simulink model "SixDOFSim"  (R2026b)
settings: Solver=VariableStepAuto  StopTime=400
values from neighbouring files (symbols this model uses):
  A = [A_1 zeros(n/2,n/2);zeros(n/2,n/2) A_2]    [defineABC.m]    (also in implicit_linmod.m = -inv(E)*A_prime; nonlinear_6DOF.m = q_d*S*CA; normieren.m = Tx\A*Tx)
  B = [B_1, zeros(n/2,m/2);zeros(n/2,m/2), B_2]    [defineABC.m]    (also in implicit_linmod.m = -inv(E)*B_prime; normieren.m = Tx\B*Tu)
  C = zeros(m,n)    [defineABC.m]    (also in normieren.m = (Ty\C*Tx))
  eta_max = 10*pi/180    (= 0.174532925199)    [SixDOFModel.m]
  eta_min = - 25*pi/180    (= -0.436332312999)    [SixDOFModel.m]
  F = -inv(C*(Ak\B))    [SixDOFModel.m]    (also in coupling_controller.m = Kopt{end}; implicit_linmod.m = feval(fun, dX_ap, X_ap, U_minus))
  I_inv = inv(I)    [initializeParameters.m]
  K = lqr(sys_ol,Q,R)    [SixDOFModel.m]
  latlon_init = [0;0]    [SixDOFModel.m]
  m = size(B_1,2) + size(B_2,2)    [defineABC.m]    (also in implicit_linmod.m = length(U_ap); initializeParameters.m = 120000)
  n = size(A_1,1) +size(A_2,2)    [defineABC.m]    (also in implicit_linmod.m = length(X_ap); normieren.m = size(A,2))
  Omega_init_1 = [0;0;0]    [SixDOFModel.m]
  Omega_init_2 = [0;0;0]    [SixDOFModel.m]
  P_e_init_1 = [0;0;-h_init_1]    [SixDOFModel.m]
  P_e_init_2 = [0;0;-h_init_2]    [SixDOFModel.m]
  Phi_init_1 = [0;0;0]    [SixDOFModel.m]
  Phi_init_2 = [0;0;0]    [SixDOFModel.m]
  sigmaf_max = 10*pi/180    (= 0.174532925199)    [SixDOFModel.m]
  sigmaf_min = 0.5*pi/180    (= 0.00872664625997)    [SixDOFModel.m]
  U_ap = [U_ap_1;U_ap_2]    [SixDOFModel.m]    (also in trimValues.m = Z_ap(11:14))
  U_test = [-0.12;1;0;0;-0.1;1;0;0]    [SixDOFModel.m]
  V_init_1 = [200;0;0]    [SixDOFModel.m]
  V_init_2 = [220;0;0]    [SixDOFModel.m]
  W_ap = [X_ap_1(1); X_ap_2(1); 0; 0; X_ap_1(10); X_ap_2(10); 0; 0]    [SixDOFModel.m]
  X_ap = [X_ap_1;X_ap_2]    [SixDOFModel.m]    (also in trimValues.m = Z_ap(1:10))
  X_init = [X_init_1;X_init_2]    [SixDOFModel.m]
  xi_max = 25*pi/180    (= 0.436332312999)    [SixDOFModel.m]
  xi_min = - xi_max    (= -0.436332312999)    [SixDOFModel.m]
  zita_max = 30*pi/180    (= 0.523598775598)    [SixDOFModel.m]
  zita_min = - zita_max    (= -0.523598775598)    [SixDOFModel.m]
undefined symbols (not defined in the file or in its folder): Earth, globalParameters, nonlinear_6DOF, WGS84
libraries: aerolibfltsims x38, aerolibtransform2 x6, aerolibwind2 x2, simulink x2, aerolibatmos2 x2
(part 1 of 3)
settings Model: Creator=teteu  LastModifiedBy=zhang
settings SolverCC: ZeroCrossAlgorithm=Adaptive
settings DebuggingCC: IgnoredZcDiagnostic=none  UnderSpecifiedDimensionMsg=warning
settings RTWCC: DLArmComputeVersion=19.05
settings SimscapeCC: SimscapeUseEnergyAccounting=off

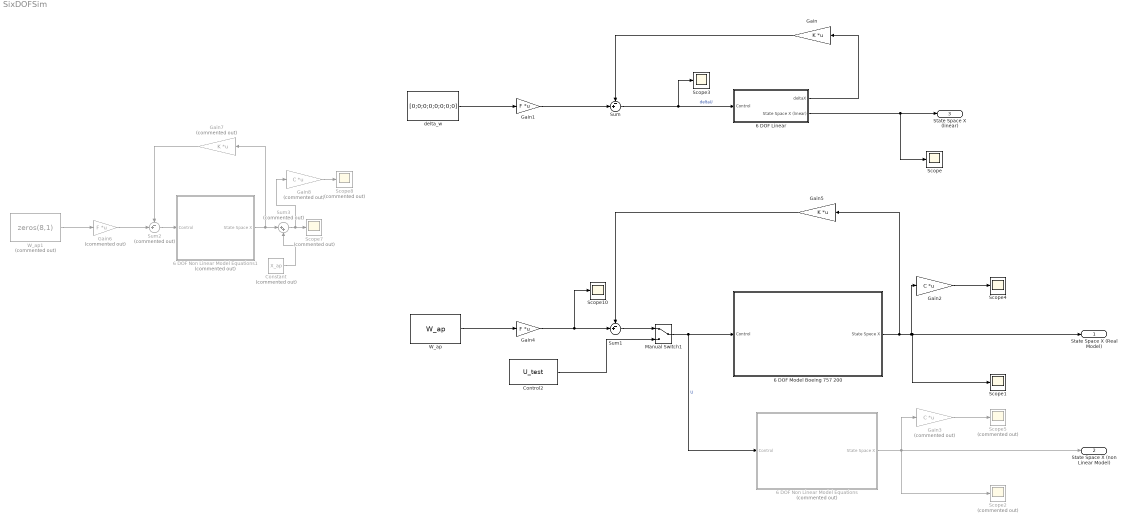
== system SixDOFSim ==
  6 DOF Linear : Subsystem
  6 DOF Model Boeing 757 200 : Subsystem
      mask Display: image('Eastern_Airlines_Boeing_757-225_N523EA_March_1990_DCW_4974892113-624x422.jpg'); % Use "Edit Image" on toolstrip to change.
  6 DOF Non Linear Model Equations : Subsystem  Commented=on
      mask Display: image('491461_1_En_8_Fig2_HTML.png');
  6 DOF Non Linear Model Equations1 : Subsystem  Commented=on
      mask Display: image('491461_1_En_8_Fig2_HTML.png');
  Constant : Constant  Commented=on  Value=X_ap
  Control2 : Constant  Value=U_test
  Gain : Gain  Gain=K  Multiplication=Matrix(K*u)
  Gain1 : Gain  Gain=F  Multiplication=Matrix(K*u)
  Gain2 : Gain  Gain=C  Multiplication=Matrix(K*u)
  Gain3 : Gain  Commented=on  Gain=C  Multiplication=Matrix(K*u)
  Gain4 : Gain  Gain=F  Multiplication=Matrix(K*u)
  Gain5 : Gain  Gain=K  Multiplication=Matrix(K*u)
  Gain6 : Gain  Commented=on  Gain=F  Multiplication=Matrix(K*u)
  Gain7 : Gain  Commented=on  Gain=K  Multiplication=Matrix(K*u)
  Gain8 : Gain  Commented=on  Gain=C  Multiplication=Matrix(K*u)
  Manual Switch1 : ManualSwitch
  Scope{,1,3..4,10} (5 alike) : Scope
      Scope settings: ActiveDisplayYMinimum=7776.65926  ActiveDisplayYMaximum=8271.84202
      Scope1 settings: ActiveDisplayYMinimum=-9243.3104191158855  ActiveDisplayYMaximum=16255.898989328776  DataLoggingVariableName=ScopeData2
      Scope10 settings: ActiveDisplayYMinimum=-20.03565  ActiveDisplayYMaximum=4.07413  DataLoggingVariableName=ScopeData6
      Scope3 settings: ActiveDisplayYMinimum=-0.10509  ActiveDisplayYMaximum=0.02343  DataLoggingVariableName=ScopeData4
      Scope4 settings: ActiveDisplayYMinimum=-2103.5512790095572  ActiveDisplayYMaximum=10071.687214697096
  Scope{2,5,7..8} (4 alike) : Scope  Commented=on
      Scope2 settings: ActiveDisplayYMinimum=-1023.1359  ActiveDisplayYMaximum=9013.89641  DataLoggingVariableName=ScopeData3
      Scope5 settings: ActiveDisplayYMinimum=-1001.29057  ActiveDisplayYMaximum=9011.46915  DataLoggingVariableName=ScopeData2
      Scope7 settings: ActiveDisplayYMinimum=-11.89027  ActiveDisplayYMaximum=4.789  DataLoggingVariableName=ScopeData4
      Scope8 settings: ActiveDisplayYMinimum=-111.74089  ActiveDisplayYMaximum=88.33649  DataLoggingVariableName=ScopeData5
  Sum : Sum  Inputs=-+|
  Sum1 : Sum  Inputs=-+|
  Sum2 : Sum  Commented=on  Inputs=-+|
  Sum3 : Sum  Commented=on  Inputs=|++
  W_ap : Constant  Value=W_ap
  W_ap1 : Constant  Commented=on  Value=zeros(8,1)
  delta_w : Constant  Value=[0;0;0;0;0;0;0;0]
  State Space X (Real Model) : Outport
  State Space X (non Linear Model) : Outport  Port=2
  State Space X (linear) : Outport  Port=3
  wires:
  Gain/1 -> Sum/1
  Sum/1 -> Scope3/1, 6 DOF Linear/1(Control)  "deltaU"
  6 DOF Linear/2(State Space X (linear)) -> Scope/1, State Space X (linear)/1
  6 DOF Model Boeing 757 200/1(State Spece X) -> Gain5/1, Gain2/1, Scope1/1, State Space X (Real Model)/1
  6 DOF Non Linear Model Equations/1(State Space X) -> Gain3/1, State Space X (non Linear Model)/1, Scope2/1
  delta_w/1 -> Gain1/1
  Gain1/1 -> Sum/2
  6 DOF Linear/1(deltaX) -> Gain/1
  Gain2/1 -> Scope4/1
  Gain3/1 -> Scope5/1
  W_ap/1 -> Gain4/1
  Gain4/1 -> Scope10/1, Sum1/2
  Gain5/1 -> Sum1/1
  Sum1/1 -> Manual Switch1/1
  Manual Switch1/1 -> 6 DOF Non Linear Model Equations/1(Control), 6 DOF Model Boeing 757 200/1(Control)  "U"
  6 DOF Non Linear Model Equations1/1(State Space X) -> Sum3/1, Gain7/1
  Sum2/1 -> 6 DOF Non Linear Model Equations1/1(Control)
  Gain7/1 -> Sum2/1
  Gain8/1 -> Scope8/1
  W_ap1/1 -> Gain6/1
  Gain6/1 -> Sum2/2
  Sum3/1 -> Gain8/1, Scope7/1
  Constant/1 -> Sum3/2
  Control2/1 -> Manual Switch1/2

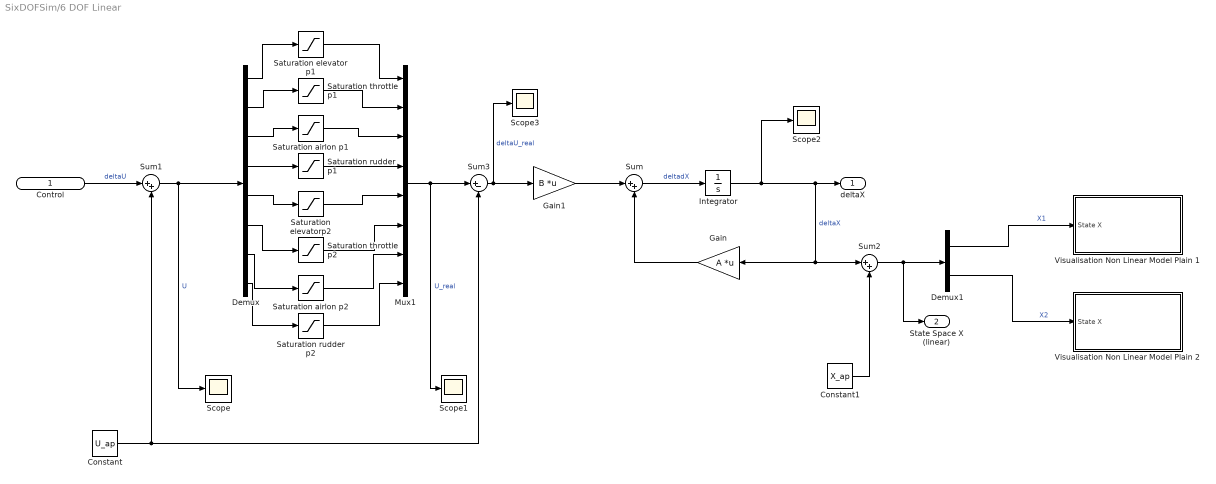
== system SixDOFSim/6 DOF Linear ==
  Control : Inport
  Constant : Constant  Value=U_ap
  Constant1 : Constant  Value=X_ap
  Demux : Demux  Outputs=8
  Demux1 : Demux  Outputs=2
  Gain : Gain  Gain=A  Multiplication=Matrix(K*u)
  Gain1 : Gain  Gain=B  Multiplication=Matrix(K*u)
  Integrator : Integrator  InitialCondition=X_init-X_ap
  Mux1 : Mux  Inputs=8
  Saturation airlon p1 : Saturate  UpperLimit=xi_max  LowerLimit=xi_min
  Saturation airlon p2 : Saturate  UpperLimit=xi_max  LowerLimit=xi_min
  Saturation elevator p1 : Saturate  UpperLimit=eta_max  LowerLimit=eta_min
  Saturation elevatorp2 : Saturate  UpperLimit=eta_max  LowerLimit=eta_min
  Saturation rudder p1 : Saturate  UpperLimit=zita_max  LowerLimit=zita_min
  Saturation rudder p2 : Saturate  UpperLimit=zita_max  LowerLimit=zita_min
  Saturation throttle p1 : Saturate  UpperLimit=sigmaf_max  LowerLimit=sigmaf_min
  Saturation throttle p2 : Saturate  UpperLimit=sigmaf_max  LowerLimit=sigmaf_min
  Scope{,1..3} (4 alike) : Scope
      Scope settings: ActiveDisplayYMinimum=-0.19857  ActiveDisplayYMaximum=0.43595  DataLoggingVariableName=ScopeData2
      Scope1 settings: ActiveDisplayYMinimum=-0.34609  ActiveDisplayYMaximum=0.23238
      Scope2 settings: ActiveDisplayYMinimum=-0.60126  ActiveDisplayYMaximum=0.68136
      Scope3 settings: ActiveDisplayYMinimum=-0.00918  ActiveDisplayYMaximum=0.00122  DataLoggingVariableName=ScopeData2
  Sum : Sum  Inputs=|++
  Sum1 : Sum  Inputs=|++
  Sum2 : Sum  Inputs=|++
  Sum3 : Sum  Inputs=|+-
  Visualisation Non Linear Model Plain 1 : Subsystem
  Visualisation Non Linear Model Plain 2 : Subsystem
  deltaX : Outport
  State Space X (linear) : Outport  Port=2
  wires:
  Gain1/1 -> Sum/1
  Sum/1 -> Integrator/1  "deltadX"
  Gain/1 -> Sum/2
  Demux/2 -> Saturation throttle p1/1
  Demux/3 -> Saturation airlon p1/1
  Demux/1 -> Saturation elevator p1/1
  Saturation elevator p1/1 -> Mux1/1
  Saturation throttle p1/1 -> Mux1/2
  Saturation airlon p1/1 -> Mux1/3
  Saturation rudder p1/1 -> Mux1/4
  Demux/4 -> Saturation rudder p1/1
  Control/1 -> Sum1/1  "deltaU"
  Constant/1 -> Sum1/2, Sum3/2
  Integrator/1 -> Scope2/1, deltaX/1, Sum2/1, Gain/1  "deltaX"
  Demux1/1 -> Visualisation Non Linear Model Plain 1/1(State X)  "X1"
  Demux1/2 -> Visualisation Non Linear Model Plain 2/1(State X)  "X2"
  Demux/5 -> Saturation elevatorp2/1
  Saturation elevatorp2/1 -> Mux1/5
  Demux/6 -> Saturation throttle p2/1
  Demux/7 -> Saturation airlon p2/1
  Saturation throttle p2/1 -> Mux1/6
  Saturation airlon p2/1 -> Mux1/7
  Demux/8 -> Saturation rudder p2/1
  Saturation rudder p2/1 -> Mux1/8
  Sum1/1 -> Demux/1, Scope/1  "U"
  Mux1/1 -> Sum3/1, Scope1/1  "U_real"
  Sum2/1 -> State Space X (linear)/1, Demux1/1
  Constant1/1 -> Sum2/2
  Sum3/1 -> Scope3/1, Gain1/1  "deltaU_real"

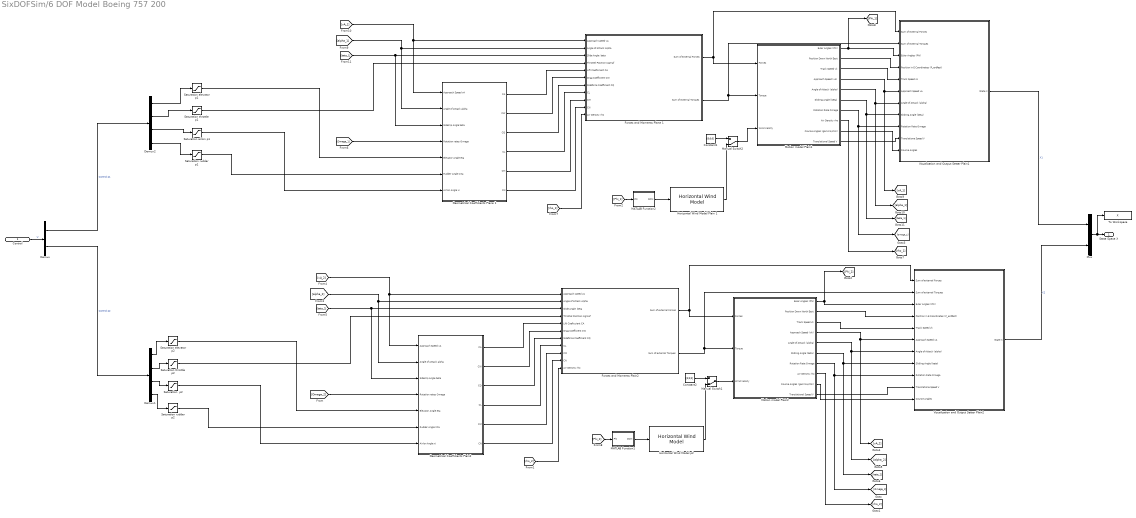
== system SixDOFSim/6 DOF Model Boeing 757 200 ==
  Control : Inport
  Constant1 : Constant  Value=[0;0;0]
  Constant2 : Constant  Value=[0;0;0]
  Demux : Demux  Outputs=2
  Demux1 : Demux
  Demux2 : Demux
  Forces and Moments Plain2 : Subsystem
  Forces and Moments Plane 1 : Subsystem
  Geometrical Coefficients Plain2 : Subsystem
  Geometrical Coefficients Plane 1 : Subsystem
  Horizontal Wind Model Plain 1 : aerolibwind2/Horizontal Wind Model  units=Metric (MKS)  Vw_source=Internal  Vwind=15  W_source=Internal  Wdeg=0
  Horizontal Wind Model p2 : aerolibwind2/Horizontal Wind Model  units=Metric (MKS)  Vw_source=Internal  Vwind=15  W_source=Internal  Wdeg=0
  MATLAB Function1 : MATLAB Function  TreatAsAtomicUnit=on
  MATLAB Function2 : MATLAB Function  TreatAsAtomicUnit=on
  Manual Switch1 : ManualSwitch  CurrentSetting=0
  Manual Switch2 : ManualSwitch  CurrentSetting=0
  Motion model Plain1 : Subsystem
  "Motion model Plain2 " : Subsystem
  Mux : Mux  Inputs=2
  Saturation  p2 : Saturate  UpperLimit=xi_max  LowerLimit=xi_min
  Saturation airlon p1 : Saturate  UpperLimit=xi_max  LowerLimit=xi_min
  Saturation elevator p1 : Saturate  UpperLimit=eta_max  LowerLimit=eta_min
  Saturation elevator p2 : Saturate  UpperLimit=eta_max  LowerLimit=eta_min
  Saturation rudder p1 : Saturate  UpperLimit=zita_max  LowerLimit=zita_min
  Saturation rudder p2 : Saturate  UpperLimit=zita_max  LowerLimit=zita_min
  Saturation throttle p1 : Saturate  UpperLimit=sigmaf_max  LowerLimit=sigmaf_min
  Saturation throttle p2 : Saturate  UpperLimit=sigmaf_max  LowerLimit=sigmaf_min
  To Workspace : ToWorkspace  VariableName=X  SaveFormat=Timeseries  SampleTime=-1
  Visualization and Output Setter Plain1 : Subsystem
  Visualization and Output Setter Plain2 : Subsystem
  State Spece X : Outport
  wires:
  "Motion model Plain2 "/7(Rotation Rate Omega) -> [Omega_2], Visualization and Output Setter Plain2/9(Rotation Rate Omega)
  "Motion model Plain2 "/3(Track Speed vk) -> Visualization and Output Setter Plain2/5(Track Speed vk)
  Visualization and Output Setter Plain2/1(State X) -> Mux/2  "X2"
  "Motion model Plain2 "/6(Slidiing Angle (beta)) -> [beta_2], Visualization and Output Setter Plain2/8(Slidiing Angle (beta))
  Forces and Moments Plain2/2(Sum of external Torques) -> Visualization and Output Setter Plain2/2(Sum of external Torques), "Motion model Plain2 "/2(Torque)
  [alpha_2] -> Geometrical Coefficients Plain2/2(Angle of Attack alpha), Forces and Moments Plain2/2(Angle of Attack Alpha)
  "Motion model Plain2 "/4(Approach Speed (vA)) -> [vA_2], Visualization and Output Setter Plain2/6(Approach Speed vA)
  Geometrical Coefficients Plain2/4(CL) -> Forces and Moments Plain2/8(CL)
  Geometrical Coefficients Plain2/1(CA) -> Forces and Moments Plain2/5(Lift Coeficcient CA)
  Forces and Moments Plain2/1(Sum of external Forces) -> Visualization and Output Setter Plain2/1(Sum of external Forces), "Motion model Plain2 "/1(Forces)
  "Motion model Plain2 "/5(Angle of Attack (alpha)) -> [alpha_2], Visualization and Output Setter Plain2/7(Angle of Attack (alpha))
  "Motion model Plain2 "/2(Position Down North East) -> Visualization and Output Setter Plain2/4(Position in E Coordinates (P_erdfest))
  "Motion model Plain2 "/1(Euler Angles (Phi)) -> [Phi_2], Visualization and Output Setter Plain2/3(Euler Angles (Phi))
  [vA_2] -> Geometrical Coefficients Plain2/1(Approach Speed vA), Forces and Moments Plain2/1(Approach speed vA)
  Geometrical Coefficients Plain2/5(CM) -> Forces and Moments Plain2/9(CM)
  Saturation  p2/1 -> Geometrical Coefficients Plain2/7(Airlon Angle xi)
  [Omega_2] -> Geometrical Coefficients Plain2/4(Rotation rates Omega)
  Saturation throttle p2/1 -> Forces and Moments Plain2/4(Throttel Position sigmaf)
  [beta_2] -> Geometrical Coefficients Plain2/3(Sideslip Angle beta), Forces and Moments Plain2/3(Slide Angle  beta)
  Geometrical Coefficients Plain2/6(CN) -> Forces and Moments Plain2/10(CN)
  "Motion model Plain2 "/8(Air Density rho) -> [rho_2]
  [rho_2] -> Forces and Moments Plain2/11(Air Density rho)
  Saturation elevator p2/1 -> Geometrical Coefficients Plain2/5(Elevator Angle eta)
  Saturation rudder p2/1 -> Geometrical Coefficients Plain2/6(Rudder Angle zita)
  Geometrical Coefficients Plain2/3(CQ) -> Forces and Moments Plain2/7(Sideforce Coefficient CQ)
  Geometrical Coefficients Plain2/2(CW) -> Forces and Moments Plain2/6(Drag Coefficient CW)
  Demux1/2 -> Saturation throttle p2/1
  Demux1/3 -> Saturation  p2/1
  Demux1/1 -> Saturation elevator p2/1
  Demux1/4 -> Saturation rudder p2/1
  "Motion model Plain2 "/9("Course Angles (gamma;chsi) ") -> Visualization and Output Setter Plain2/11("Course Angles ")
  "Motion model Plain2 "/10(Translational Speed V) -> Visualization and Output Setter Plain2/10(Translationa Speed V)
  Manual Switch1/1 -> "Motion model Plain2 "/3(Wind Veloity)
  Saturation rudder p1/1 -> Geometrical Coefficients Plane 1/6(Rudder Angle zita)
  Motion model Plain1/5(Angle of Attack (alpha)) -> [alpha_1], Visualization and Output Setter Plain1/7(Angle of Attack (alpha))
  Motion model Plain1/1(Euler Angles (Phi)) -> [Phi_1], Visualization and Output Setter Plain1/3(Euler Angles (Phi))
  Forces and Moments Plane 1/1(Sum of external Forces) -> Visualization and Output Setter Plain1/1(Sum of external Forces), Motion model Plain1/1(Forces)
  Motion model Plain1/10(Translational Speed V) -> Visualization and Output Setter Plain1/10(Translationa Speed V)
  [Omega_1] -> Geometrical Coefficients Plane 1/4(Rotation rates Omega)
  Geometrical Coefficients Plane 1/2(CW) -> Forces and Moments Plane 1/6(Drag Coefficient CW)
  [beta_1] -> Geometrical Coefficients Plane 1/3(Sideslip Angle beta), Forces and Moments Plane 1/3(Slide Angle  beta)
  Geometrical Coefficients Plane 1/3(CQ) -> Forces and Moments Plane 1/7(Sideforce Coefficient CQ)
  Geometrical Coefficients Plane 1/4(CL) -> Forces and Moments Plane 1/8(CL)
  Saturation airlon p1/1 -> Geometrical Coefficients Plane 1/7(Airlon Angle xi)
  Geometrical Coefficients Plane 1/5(CM) -> Forces and Moments Plane 1/9(CM)
  Motion model Plain1/4(Approach Speed (vA)) -> [vA_1], Visualization and Output Setter Plain1/6(Approach Speed vA)
  Demux2/3 -> Saturation airlon p1/1
  [vA_1] -> Geometrical Coefficients Plane 1/1(Approach Speed vA), Forces and Moments Plane 1/1(Approach speed vA)
  Saturation throttle p1/1 -> Forces and Moments Plane 1/4(Throttel Position sigmaf)
  Demux2/1 -> Saturation elevator p1/1
  Motion model Plain1/2(Position Down North East) -> Visualization and Output Setter Plain1/4(Position in E Coordinates (P_erdfest))
  Geometrical Coefficients Plane 1/1(CA) -> Forces and Moments Plane 1/5(Lift Coeficcient CA)
  Demux2/2 -> Saturation throttle p1/1
  Motion model Plain1/8(Air Density rho) -> [rho_1]
  [rho_1] -> Forces and Moments Plane 1/11(Air Density rho)
  Motion model Plain1/6(Slidiing Angle (beta)) -> [beta_1], Visualization and Output Setter Plain1/8(Slidiing Angle (beta))
  Demux2/4 -> Saturation rudder p1/1
  Motion model Plain1/9("Course Angles (gamma;chsi) ") -> Visualization and Output Setter Plain1/11("Course Angles ")
  Motion model Plain1/7(Rotation Rate Omega) -> [Omega_1], Visualization and Output Setter Plain1/9(Rotation Rate Omega)
  Saturation elevator p1/1 -> Geometrical Coefficients Plane 1/5(Elevator Angle eta)
  Forces and Moments Plane 1/2(Sum of external Torques) -> Visualization and Output Setter Plain1/2(Sum of external Torques), Motion model Plain1/2(Torque)
  [alpha_1] -> Geometrical Coefficients Plane 1/2(Angle of Attack alpha), Forces and Moments Plane 1/2(Angle of Attack Alpha)
  Geometrical Coefficients Plane 1/6(CN) -> Forces and Moments Plane 1/10(CN)
  Motion model Plain1/3(Track Speed vk) -> Visualization and Output Setter Plain1/5(Track Speed vk)
  Visualization and Output Setter Plain1/1(State X) -> Mux/1  "X1"
  [Phi_2] -> MATLAB Function1/1(Phi)
  Horizontal Wind Model p2/1 -> Manual Switch1/2
  MATLAB Function1/1(DCM) -> Horizontal Wind Model p2/1
  Control/1 -> Demux/1  "U"
  Demux/1 -> Demux2/1  "Control p1"
  Demux/2 -> Demux1/1  "Control p2"
  Constant2/1 -> Manual Switch1/1
  MATLAB Function2/1(DCM) -> Horizontal Wind Model Plain 1/1
  [Phi_1] -> MATLAB Function2/1(Phi)
  Constant1/1 -> Manual Switch2/1
  Horizontal Wind Model Plain 1/1 -> Manual Switch2/2
  Manual Switch2/1 -> Motion model Plain1/3(Wind Veloity)
  Mux/1 -> To Workspace/1, State Spece X/1

== system SixDOFSim/6 DOF Non Linear Model Equations ==
  Control : Inport
  Demux : Demux
  Demux1 : Demux
  Demux2 : Demux  Outputs=2
  Integrator : Integrator  InitialCondition=X_init(1:n/2)
  Integrator1 : Integrator  InitialCondition=X_init(1+n/2:end)
  Model of the Plain Equations 1 : MATLABFcn  MATLABFcn=nonlinear_6DOF(u(1:10),u(11:14),u(15))
  Model of the Plain Equations 2 : MATLABFcn  MATLABFcn=nonlinear_6DOF(u(1:10),u(11:14),u(15))
  Mux : Mux  Inputs=3
  Mux1 : Mux
  Mux2 : Mux  Inputs=3
  Mux3 : Mux
  Mux4 : Mux  Inputs=2
  Mux5 : Mux  Inputs=2
  Saturation airlon p1 : Saturate  UpperLimit=xi_max  LowerLimit=xi_min
  Saturation airlonp2 : Saturate  UpperLimit=xi_max  LowerLimit=xi_min
  Saturation elevator p1 : Saturate  UpperLimit=eta_max  LowerLimit=eta_min
  Saturation elevator p2 : Saturate  UpperLimit=eta_max  LowerLimit=eta_min
  Saturation rudder p1 : Saturate  UpperLimit=zita_max  LowerLimit=zita_min
  Saturation rudder p2 : Saturate  UpperLimit=zita_max  LowerLimit=zita_min
  Saturation throttle p1 : Saturate  UpperLimit=sigmaf_max  LowerLimit=sigmaf_min
  Saturation throttle p2 : Saturate  UpperLimit=sigmaf_max  LowerLimit=sigmaf_min
  Scope : Scope
      settings: ActiveDisplayYMinimum=-0.40615  ActiveDisplayYMaximum=0.92239  DataLoggingVariableName=ScopeData3
  Scope1 : Scope
      settings: ActiveDisplayYMinimum=-0.28294  ActiveDisplayYMaximum=0.22359  DataLoggingVariableName=ScopeData4
  Select Plain 1 : Constant
  Select Plain 2 : Constant  Value=2
  Visualisation Non Linear Model 1 : Subsystem
  Visualisation Non Linear Model 2 : Subsystem  Commented=on
  State Space X : Outport
  wires:
  Model of the Plain Equations 1/1 -> Integrator/1  "dX"
  Integrator/1 -> Visualisation Non Linear Model 1/1(State X), Mux/1, Mux4/1  "X1"
  Mux/1 -> Model of the Plain Equations 1/1
  Demux/1 -> Saturation elevator p1/1
  Demux/2 -> Saturation throttle p1/1
  Demux/3 -> Saturation airlon p1/1
  Demux/4 -> Saturation rudder p1/1
  Saturation elevator p1/1 -> Mux1/1
  Saturation throttle p1/1 -> Mux1/2
  Saturation airlon p1/1 -> Mux1/3
  Saturation rudder p1/1 -> Mux1/4
  Mux1/1 -> Mux5/1, Mux/2  "Control Plain 1"
  Mux2/1 -> Model of the Plain Equations 2/1
  Integrator1/1 -> Visualisation Non Linear Model 2/1(State X), Mux4/2, Mux2/1  "X2"
  Mux3/1 -> Mux2/2, Mux5/2  "Control P2"
  Saturation rudder p2/1 -> Mux3/4
  Saturation throttle p2/1 -> Mux3/2
  Saturation elevator p2/1 -> Mux3/1
  Demux2/2 -> Demux1/1
  Saturation airlonp2/1 -> Mux3/3
  Demux1/1 -> Saturation elevator p2/1
  Demux1/3 -> Saturation airlonp2/1
  Demux1/4 -> Saturation rudder p2/1
  Demux1/2 -> Saturation throttle p2/1
  Model of the Plain Equations 2/1 -> Integrator1/1  "dX"
  Control/1 -> Scope/1, Demux2/1
  Demux2/1 -> Demux/1
  Mux4/1 -> State Space X/1
  Select Plain 1/1 -> Mux/3
  Select Plain 2/1 -> Mux2/3
  Mux5/1 -> Scope1/1

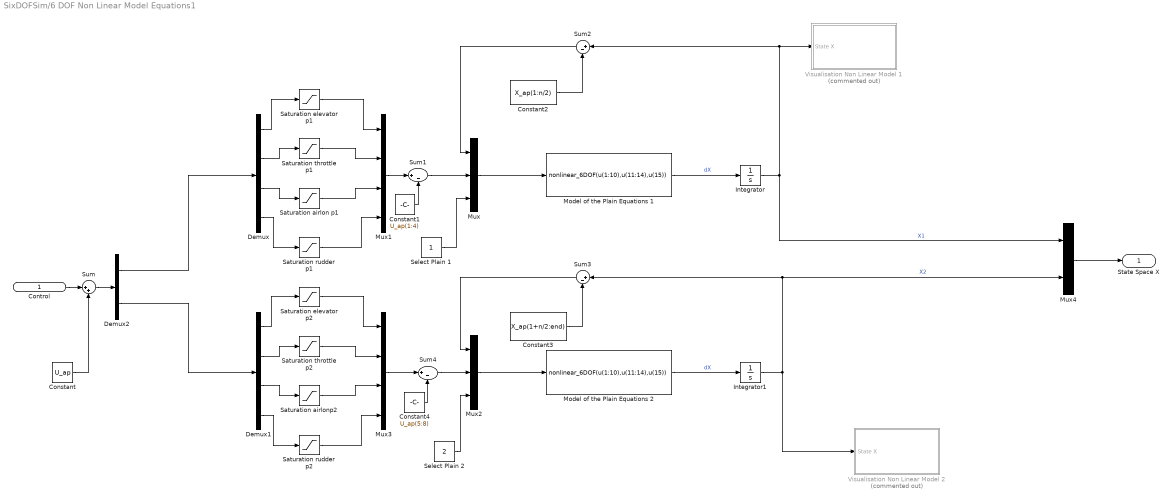
== system SixDOFSim/6 DOF Non Linear Model Equations1 ==
  Control : Inport
  Constant : Constant  Value=U_ap
  Constant1 : Constant  Value=U_ap(1:4)
  Constant2 : Constant  Value=X_ap(1:n/2)
  Constant3 : Constant  Value=X_ap(1+n/2:end)
  Constant4 : Constant  Value=U_ap(5:8)
  Demux : Demux
  Demux1 : Demux
  Demux2 : Demux  Outputs=2
  Integrator : Integrator  InitialCondition=X_init(1:n/2)-X_ap(1:n/2)
  Integrator1 : Integrator  InitialCondition=X_init(1+n/2:end)-X_ap(1+n/2:end)
  Model of the Plain Equations 1 : MATLABFcn  MATLABFcn=nonlinear_6DOF(u(1:10),u(11:14),u(15))
  Model of the Plain Equations 2 : MATLABFcn  MATLABFcn=nonlinear_6DOF(u(1:10),u(11:14),u(15))
  Mux : Mux  Inputs=3
  Mux1 : Mux
  Mux2 : Mux  Inputs=3
  Mux3 : Mux
  Mux4 : Mux  Inputs=2
  Saturation airlon p1 : Saturate  UpperLimit=xi_max  LowerLimit=xi_min
  Saturation airlonp2 : Saturate  UpperLimit=xi_max  LowerLimit=xi_min
  Saturation elevator p1 : Saturate  UpperLimit=eta_max  LowerLimit=eta_min
  Saturation elevator p2 : Saturate  UpperLimit=eta_max  LowerLimit=eta_min
  Saturation rudder p1 : Saturate  UpperLimit=zita_max  LowerLimit=zita_min
  Saturation rudder p2 : Saturate  UpperLimit=zita_max  LowerLimit=zita_min
  Saturation throttle p1 : Saturate  UpperLimit=sigmaf_max  LowerLimit=sigmaf_min
  Saturation throttle p2 : Saturate  UpperLimit=sigmaf_max  LowerLimit=sigmaf_min
  Select Plain 1 : Constant
  Select Plain 2 : Constant  Value=2
  Sum : Sum  Inputs=|++
  Sum{1..4} (4 alike) : Sum  Inputs=|+-
  Visualisation Non Linear Model 1 : Subsystem  Commented=on
  Visualisation Non Linear Model 2 : Subsystem  Commented=on
  State Space X : Outport
  wires:
  Model of the Plain Equations 1/1 -> Integrator/1  "dX"
  Integrator/1 -> Visualisation Non Linear Model 1/1(State X), Sum2/1, Mux4/1  "X1"
  Mux/1 -> Model of the Plain Equations 1/1
  Demux/1 -> Saturation elevator p1/1
  Demux/2 -> Saturation throttle p1/1
  Demux/3 -> Saturation airlon p1/1
  Demux/4 -> Saturation rudder p1/1
  Saturation elevator p1/1 -> Mux1/1
  Saturation throttle p1/1 -> Mux1/2
  Saturation airlon p1/1 -> Mux1/3
  Saturation rudder p1/1 -> Mux1/4
  Mux2/1 -> Model of the Plain Equations 2/1
  Integrator1/1 -> Visualisation Non Linear Model 2/1(State X), Mux4/2, Sum3/1  "X2"
  Saturation rudder p2/1 -> Mux3/4
  Saturation throttle p2/1 -> Mux3/2
  Saturation elevator p2/1 -> Mux3/1
  Demux2/2 -> Demux1/1
  Saturation airlonp2/1 -> Mux3/3
  Demux1/1 -> Saturation elevator p2/1
  Demux1/3 -> Saturation airlonp2/1
  Demux1/4 -> Saturation rudder p2/1
  Demux1/2 -> Saturation throttle p2/1
  Model of the Plain Equations 2/1 -> Integrator1/1  "dX"
  Demux2/1 -> Demux/1
  Mux4/1 -> State Space X/1
  Select Plain 1/1 -> Mux/3
  Select Plain 2/1 -> Mux2/3
  Sum/1 -> Demux2/1
  Control/1 -> Sum/1
  Constant/1 -> Sum/2
  Sum1/1 -> Mux/2
  Mux1/1 -> Sum1/1
  Constant1/1 -> Sum1/2
  Sum2/1 -> Mux/1
  Constant2/1 -> Sum2/2
  Constant3/1 -> Sum3/2
  Sum3/1 -> Mux2/1
  Sum4/1 -> Mux2/2
  Constant4/1 -> Sum4/2
  Mux3/1 -> Sum4/1

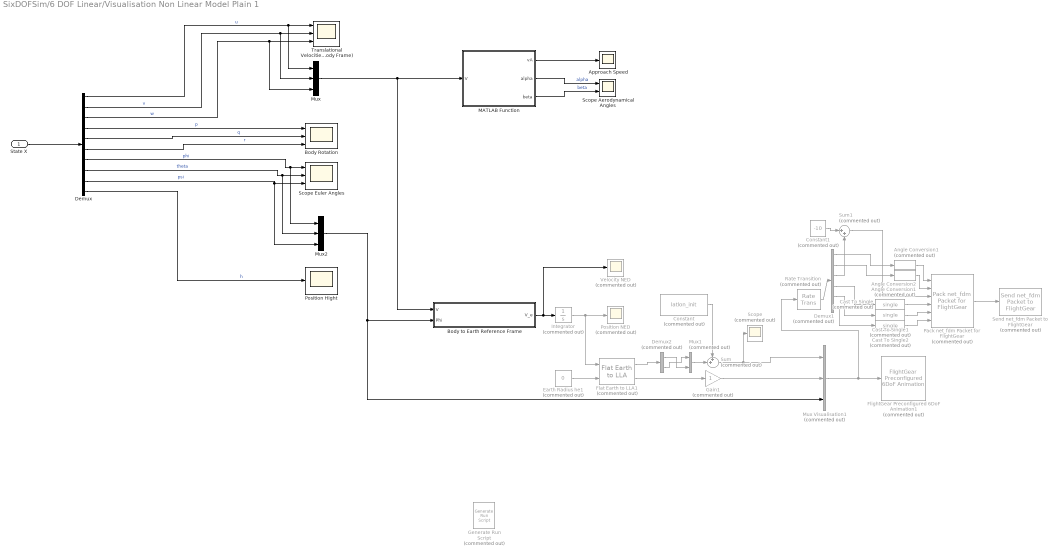
== system SixDOFSim/6 DOF Linear/Visualisation Non Linear Model Plain 1 ==
  State X : Inport
  Angle Conversion1 : aerolibfltsims/FlightGear Preconfigured 6DoF Animation/Angle Conversion1  Commented=on  SystemSampleTime=-1  VariantActivationTime=update diagram  Latency=0  AutoFrameSizeCalculation=off
  Angle Conversion2 : aerolibfltsims/FlightGear Preconfigured 6DoF Animation/Angle Conversion1  Commented=on  SystemSampleTime=-1  VariantActivationTime=update diagram  Latency=0  AutoFrameSizeCalculation=off
  Approach Speed : Scope
      settings: ActiveDisplayYMinimum=91.83935  ActiveDisplayYMaximum=100.90674  DataLoggingVariableName=ScopeData5
  Body Rotation : Scope  NumInputPorts=3
      settings: ActiveDisplayYMinimum=-0.01296  ActiveDisplayYMaximum=0.00254  DataLoggingVariableName=ScopeData4
  "Body to Earth Reference Frame " : MATLAB Function  TreatAsAtomicUnit=on
  Cast To Single : DataTypeConversion  Commented=on  OutDataTypeStr=single  SaturateOnIntegerOverflow=off  RndMeth=Floor
  Cast To Single1 : DataTypeConversion  Commented=on  OutDataTypeStr=single  SaturateOnIntegerOverflow=off  RndMeth=Floor
  Cast To Single2 : DataTypeConversion  Commented=on  OutDataTypeStr=single  SaturateOnIntegerOverflow=off  RndMeth=Floor
  Constant : Constant  Commented=on  Value=latlon_init
  Constant1 : Constant  Commented=on  Value=-10
  Demux : Demux  Outputs=10
  Demux1 : Demux  Commented=on  Outputs=6
  Demux2 : Demux  Commented=on  Outputs=2
  Earth Radius he1 : Constant  Commented=on  Value=0
  Flat Earth to LLA1 : aerolibtransform2/Flat Earth to LLA  Commented=on  units=Metric (MKS)  ptype=Earth (WGS84)  F=1/298.257223563  R=6378137  refPosPort=off  LL0=[0 10]  psi=0
  FlightGear Preconfigured 6DoF Animation1 : aerolibfltsims/FlightGear Preconfigured 6DoF Animation  Commented=on  xFlightGearVersion=v2019.1  DestinationIpAddress=127.0.0.1  DestinationPort=5502  SampleTime=1/30  packetVersion=24
  Gain1 : Gain  Commented=on
  Generate Run Script : aerolibfltsims/Generate Run Script  Commented=on  Architecture=Win64  dataFlow=Send  GeometryModelName=c172p  AirportId=KSFO  RunwayId=10L  InitialAltitude=7224  InitialHeading=113  OffsetDistance=4.72  OffsetAzimuth=0  InstallScenery=off  DisableShaders=on  OriginAddress=127.0.0.1  DestinationPort=5502  OriginPort=5505  LocalAddress=127.0.0.1  OutputFileName=runfg.bat  FlightGearBaseDirectory=D:\Flight Gear\FlightGear 2018.1.1
  Integrator : Integrator  Commented=on  InitialCondition=P_e_init_1
  MATLAB Function : MATLAB Function  TreatAsAtomicUnit=on
  Mux : Mux  Inputs=3
  Mux Visualisation1 : Mux  Commented=on  Inputs=3
  Mux1 : Mux  Commented=on  Inputs=2
  Mux2 : Mux  Inputs=3
  Pack net_fdm Packet for FlightGear : aerolibfltsims/Pack net_fdm Packet for FlightGear  Commented=on  FlightGearVersion=v2019.1  ShowPositionAttitudeInputs=on  ShowVelocityAccelerationInputs=off  ShowControlSurfacePositionInputs=off  ShowEngineFuelInputs=off  ShowLandingGearInputs=off  ShowEnvironmentInputs=off  SampleTime=1/30  packetVersion=24
  Position Hight : Scope
      settings: ActiveDisplayYMinimum=987.27721  ActiveDisplayYMaximum=1076.40239  DataLoggingVariableName=ScopeData2
  Position NED : Scope  Commented=on
      settings: ActiveDisplayYMinimum=-1768.43643  ActiveDisplayYMaximum=5644.14859
  Rate Transition : RateTransition  Commented=on  Integrity=off  Deterministic=off
  Scope : Scope  Commented=on
      settings: ActiveDisplayYMinimum=9.99999999993  ActiveDisplayYMaximum=10.00000000031  DataLoggingVariableName=ScopeData7
  Scope Aerodynamical Angles : Scope  NumInputPorts=2
      settings: ActiveDisplayYMinimum=-0.03275  ActiveDisplayYMaximum=0.00367
  Scope Euler Angles : Scope  NumInputPorts=3
      settings: ActiveDisplayYMinimum=-0.02717  ActiveDisplayYMaximum=0.00313  DataLoggingVariableName=ScopeData3
  Send net_fdm Packet to FlightGear : aerolibfltsims/Send net_fdm Packet to FlightGear  Commented=on  DestinationIpAddress=127.0.0.1  DestinationPort=5503  LocalIpPort=-1  varLen=off  SampleTime=1/30
  Sum : Sum  Commented=on  Inputs=++|
  Sum1 : Sum  Commented=on  Inputs=|++
  Translational Velocities (Body Frame) : Scope  NumInputPorts=3
      settings: ActiveDisplayYMinimum=-16.60398  ActiveDisplayYMaximum=149.73097
  Velocity NED : Scope  Commented=on
      settings: ActiveDisplayYMinimum=-17.2392  ActiveDisplayYMaximum=95.69716  DataLoggingVariableName=ScopeData2
  wires:
  State X/1 -> Demux/1
  Demux2/2 -> Mux1/1
  Flat Earth to LLA1/2 -> Gain1/1
  Gain1/1 -> Mux Visualisation1/2
  Mux Visualisation1/1 -> FlightGear Preconfigured 6DoF Animation1/1, Rate Transition/1
  Earth Radius he1/1 -> Flat Earth to LLA1/2
  Flat Earth to LLA1/1 -> Demux2/1
  Demux2/1 -> Mux1/2
  "Body to Earth Reference Frame "/1(V_e) -> Velocity NED/1, Integrator/1
  Integrator/1 -> Position NED/1, Flat Earth to LLA1/1
  Demux/1 -> Mux/1, Translational Velocities (Body Frame)/1  "u"
  Demux/2 -> Mux/2, Translational Velocities (Body Frame)/2  "v"
  Demux/3 -> Translational Velocities (Body Frame)/3, Mux/3  "w"
  Demux/4 -> Body Rotation/1  "p"
  Demux/5 -> Body Rotation/2  "q"
  Demux/6 -> Body Rotation/3  "r"
  Demux/7 -> Mux2/1, Scope Euler Angles/1  "phi"
  Demux/8 -> Mux2/2, Scope Euler Angles/2  "theta"
  Demux/9 -> Mux2/3, Scope Euler Angles/3  "psi"
  Demux/10 -> Position Hight/1  "h"
  Mux/1 -> MATLAB Function/1(V), "Body to Earth Reference Frame "/1(V)
  Mux2/1 -> "Body to Earth Reference Frame "/2(Phi), Mux Visualisation1/3
  MATLAB Function/1(vA) -> Approach Speed/1
  MATLAB Function/2(alpha) -> Scope Aerodynamical Angles/1  "alpha"
  MATLAB Function/3(beta) -> Scope Aerodynamical Angles/2  "beta"
  Mux1/1 -> Sum/2
  Sum/1 -> Scope/1, Mux Visualisation1/1
  Constant/1 -> Sum/1
  Pack net_fdm Packet for FlightGear/1 -> Send net_fdm Packet to FlightGear/1
  Angle Conversion1/1 -> Pack net_fdm Packet for FlightGear/1
  Angle Conversion2/1 -> Pack net_fdm Packet for FlightGear/2
  Cast To Single/1 -> Pack net_fdm Packet for FlightGear/4
  Cast To Single1/1 -> Pack net_fdm Packet for FlightGear/5
  Cast To Single2/1 -> Pack net_fdm Packet for FlightGear/6
  Demux1/2 -> Angle Conversion2/1
  Rate Transition/1 -> Demux1/1
  Demux1/1 -> Angle Conversion1/1
  Constant1/1 -> Sum1/1
  Demux1/3 -> Sum1/2
  Sum1/1 -> Pack net_fdm Packet for FlightGear/3
  Demux1/4 -> Cast To Single/1
  Demux1/5 -> Cast To Single1/1
  Demux1/6 -> Cast To Single2/1

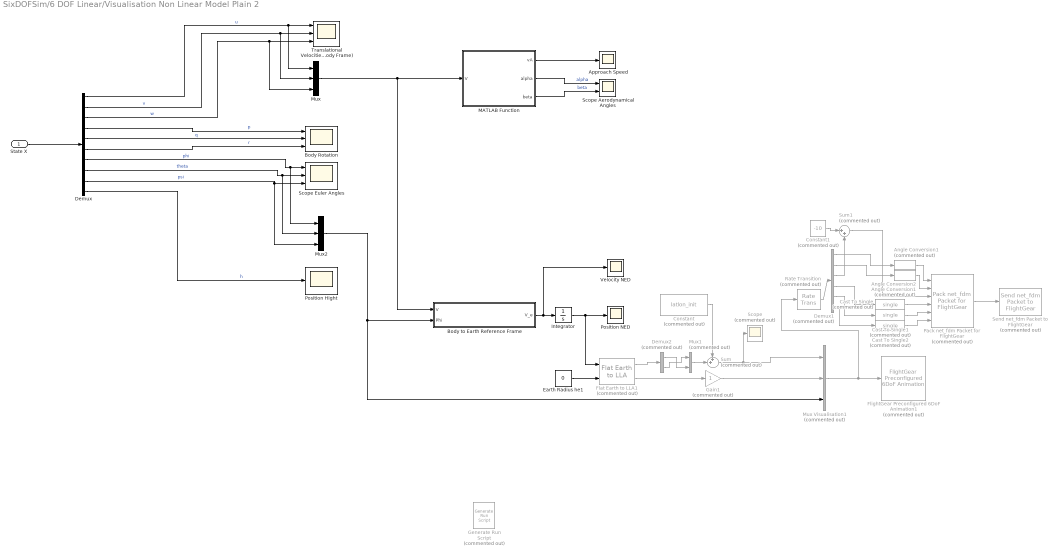
== system SixDOFSim/6 DOF Linear/Visualisation Non Linear Model Plain 2 ==
  State X : Inport
  Angle Conversion1 : aerolibfltsims/FlightGear Preconfigured 6DoF Animation/Angle Conversion1  Commented=on  SystemSampleTime=-1  VariantActivationTime=update diagram  Latency=0  AutoFrameSizeCalculation=off
  Angle Conversion2 : aerolibfltsims/FlightGear Preconfigured 6DoF Animation/Angle Conversion1  Commented=on  SystemSampleTime=-1  VariantActivationTime=update diagram  Latency=0  AutoFrameSizeCalculation=off
  Approach Speed : Scope
      settings: ActiveDisplayYMinimum=90.717446245698  ActiveDisplayYMaximum=90.71744624575  DataLoggingVariableName=ScopeData5
  Body Rotation : Scope  NumInputPorts=3
      settings: ActiveDisplayYMinimum=-4.9E-13  ActiveDisplayYMaximum=1.7E-13  DataLoggingVariableName=ScopeData4
  "Body to Earth Reference Frame " : MATLAB Function  TreatAsAtomicUnit=on
  Cast To Single : DataTypeConversion  Commented=on  OutDataTypeStr=single  SaturateOnIntegerOverflow=off  RndMeth=Floor
  Cast To Single1 : DataTypeConversion  Commented=on  OutDataTypeStr=single  SaturateOnIntegerOverflow=off  RndMeth=Floor
  Cast To Single2 : DataTypeConversion  Commented=on  OutDataTypeStr=single  SaturateOnIntegerOverflow=off  RndMeth=Floor
  Constant : Constant  Commented=on  Value=latlon_init
  Constant1 : Constant  Commented=on  Value=-10
  Demux : Demux  Outputs=10
  Demux1 : Demux  Commented=on  Outputs=6
  Demux2 : Demux  Commented=on  Outputs=2
  Earth Radius he1 : Constant  Value=0
  Flat Earth to LLA1 : aerolibtransform2/Flat Earth to LLA  Commented=on  units=Metric (MKS)  ptype=Earth (WGS84)  F=1/298.257223563  R=6378137  refPosPort=off  LL0=[0 10]  psi=0
  FlightGear Preconfigured 6DoF Animation1 : aerolibfltsims/FlightGear Preconfigured 6DoF Animation  Commented=on  xFlightGearVersion=v2019.1  DestinationIpAddress=127.0.0.1  DestinationPort=5502  SampleTime=1/30  packetVersion=24
  Gain1 : Gain  Commented=on
  Generate Run Script : aerolibfltsims/Generate Run Script  Commented=on  Architecture=Win64  dataFlow=Send  GeometryModelName=c172p  AirportId=KSFO  RunwayId=10L  InitialAltitude=7224  InitialHeading=113  OffsetDistance=4.72  OffsetAzimuth=0  InstallScenery=off  DisableShaders=on  OriginAddress=127.0.0.1  DestinationPort=5502  OriginPort=5505  LocalAddress=127.0.0.1  OutputFileName=runfg.bat  FlightGearBaseDirectory=D:\Flight Gear\FlightGear 2018.1.1
  Integrator : Integrator  InitialCondition=P_e_init_2
  MATLAB Function : MATLAB Function  TreatAsAtomicUnit=on
  Mux : Mux  Inputs=3
  Mux Visualisation1 : Mux  Commented=on  Inputs=3
  Mux1 : Mux  Commented=on  Inputs=2
  Mux2 : Mux  Inputs=3
  Pack net_fdm Packet for FlightGear : aerolibfltsims/Pack net_fdm Packet for FlightGear  Commented=on  FlightGearVersion=v2019.1  ShowPositionAttitudeInputs=on  ShowVelocityAccelerationInputs=off  ShowControlSurfacePositionInputs=off  ShowEngineFuelInputs=off  ShowLandingGearInputs=off  ShowEnvironmentInputs=off  SampleTime=1/30  packetVersion=24
  Position Hight : Scope
      settings: ActiveDisplayYMinimum=992.69224  ActiveDisplayYMaximum=1165.76794  DataLoggingVariableName=ScopeData2
  Position NED : Scope
      settings: ActiveDisplayYMinimum=-1351.79362  ActiveDisplayYMaximum=2166.14254
  Rate Transition : RateTransition  Commented=on  Integrity=off  Deterministic=off
  Scope : Scope  Commented=on
      settings: ActiveDisplayYMinimum=9.99999999993  ActiveDisplayYMaximum=10.00000000031  DataLoggingVariableName=ScopeData7
  Scope Aerodynamical Angles : Scope  NumInputPorts=2
      settings: ActiveDisplayYMinimum=-0.00068  ActiveDisplayYMaximum=0.00608
  Scope Euler Angles : Scope  NumInputPorts=3
      settings: ActiveDisplayYMinimum=-0.025  ActiveDisplayYMaximum=0.225  DataLoggingVariableName=ScopeData3
  Send net_fdm Packet to FlightGear : aerolibfltsims/Send net_fdm Packet to FlightGear  Commented=on  DestinationIpAddress=127.0.0.1  DestinationPort=5503  LocalIpPort=-1  varLen=off  SampleTime=1/30
  Sum : Sum  Commented=on  Inputs=++|
  Sum1 : Sum  Commented=on  Inputs=|++
  Translational Velocities (Body Frame) : Scope  NumInputPorts=3
      settings: ActiveDisplayYMinimum=-38.01035  ActiveDisplayYMaximum=109.05807
  Velocity NED : Scope
      settings: ActiveDisplayYMinimum=-11.33968  ActiveDisplayYMaximum=102.05713  DataLoggingVariableName=ScopeData2
  wires:
  State X/1 -> Demux/1
  Demux2/2 -> Mux1/1
  Flat Earth to LLA1/2 -> Gain1/1
  Gain1/1 -> Mux Visualisation1/2
  Mux Visualisation1/1 -> FlightGear Preconfigured 6DoF Animation1/1, Rate Transition/1
  Earth Radius he1/1 -> Flat Earth to LLA1/2
  Flat Earth to LLA1/1 -> Demux2/1
  Demux2/1 -> Mux1/2
  "Body to Earth Reference Frame "/1(V_e) -> Velocity NED/1, Integrator/1
  Integrator/1 -> Position NED/1, Flat Earth to LLA1/1
  Demux/1 -> Mux/1, Translational Velocities (Body Frame)/1  "u"
  Demux/2 -> Mux/2, Translational Velocities (Body Frame)/2  "v"
  Demux/3 -> Translational Velocities (Body Frame)/3, Mux/3  "w"
  Demux/4 -> Body Rotation/1  "p"
  Demux/5 -> Body Rotation/2  "q"
  Demux/6 -> Body Rotation/3  "r"
  Demux/7 -> Mux2/1, Scope Euler Angles/1  "phi"
  Demux/8 -> Mux2/2, Scope Euler Angles/2  "theta"
  Demux/9 -> Mux2/3, Scope Euler Angles/3  "psi"
  Demux/10 -> Position Hight/1  "h"
  Mux/1 -> MATLAB Function/1(V), "Body to Earth Reference Frame "/1(V)
  Mux2/1 -> "Body to Earth Reference Frame "/2(Phi), Mux Visualisation1/3
  MATLAB Function/1(vA) -> Approach Speed/1
  MATLAB Function/2(alpha) -> Scope Aerodynamical Angles/1  "alpha"
  MATLAB Function/3(beta) -> Scope Aerodynamical Angles/2  "beta"
  Mux1/1 -> Sum/2
  Sum/1 -> Scope/1, Mux Visualisation1/1
  Constant/1 -> Sum/1
  Pack net_fdm Packet for FlightGear/1 -> Send net_fdm Packet to FlightGear/1
  Angle Conversion1/1 -> Pack net_fdm Packet for FlightGear/1
  Angle Conversion2/1 -> Pack net_fdm Packet for FlightGear/2
  Cast To Single/1 -> Pack net_fdm Packet for FlightGear/4
  Cast To Single1/1 -> Pack net_fdm Packet for FlightGear/5
  Cast To Single2/1 -> Pack net_fdm Packet for FlightGear/6
  Demux1/2 -> Angle Conversion2/1
  Rate Transition/1 -> Demux1/1
  Demux1/1 -> Angle Conversion1/1
  Constant1/1 -> Sum1/1
  Demux1/3 -> Sum1/2
  Sum1/1 -> Pack net_fdm Packet for FlightGear/3
  Demux1/4 -> Cast To Single/1
  Demux1/5 -> Cast To Single1/1
  Demux1/6 -> Cast To Single2/1

== system SixDOFSim/6 DOF Model Boeing 757 200/Forces and Moments Plain2 ==
  Approach speed vA : Inport
  Angle of Attack Alpha : Inport  Port=2
  Slide Angle  beta : Inport  Port=3
  Throttel Position sigmaf : Inport  Port=4
  Lift Coeficcient CA : Inport  Port=5
  Drag Coefficient CW : Inport  Port=6
  Sideforce Coefficient CQ : Inport  Port=7
  CL : Inport  Port=8
  CM : Inport  Port=9
  CN : Inport  Port=10
  Air Density rho : Inport  Port=11
  Aerodynamical Forces : MATLAB Function  TreatAsAtomicUnit=on
  Aerodynamical Forces RA : Scope
      settings: ActiveDisplayYMinimum=-5.2551272052862361E+31  ActiveDisplayYMaximum=1.1237617783015539E+32
  Aerodynamical Torque : MATLAB Function  TreatAsAtomicUnit=on
  Sum : Sum  Inputs=++|
  Sum1 : Sum  Inputs=|++
  Thrust Force and Torque : MATLAB Function  TreatAsAtomicUnit=on
  Sum of external Forces : Outport
  Sum of external Torques : Outport  Port=2
  wires:
  Aerodynamical Forces/1(RA) -> Aerodynamical Forces RA/1, Sum1/1, Aerodynamical Torque/1(RA)
  Aerodynamical Torque/1(QA) -> Sum/2
  Sum1/1 -> Sum of external Forces/1
  Sum/1 -> Sum of external Torques/1
  Throttel Position sigmaf/1 -> Thrust Force and Torque/1(sigmaf)
  Thrust Force and Torque/1(Rf) -> Sum1/2
  Thrust Force and Torque/2(Qf) -> Sum/1
  Angle of Attack Alpha/1 -> Aerodynamical Forces/5(alpha)
  Slide Angle  beta/1 -> Aerodynamical Forces/6(beta)
  Approach speed vA/1 -> Aerodynamical Forces/4(vA), Aerodynamical Torque/5(vA)
  Lift Coeficcient CA/1 -> Aerodynamical Forces/1(CA)
  Drag Coefficient CW/1 -> Aerodynamical Forces/2(CW)
  Sideforce Coefficient CQ/1 -> Aerodynamical Forces/3(CQ)
  CL/1 -> Aerodynamical Torque/2(CL)
  CM/1 -> Aerodynamical Torque/3(CM)
  CN/1 -> Aerodynamical Torque/4(CN)
  Air Density rho/1 -> Aerodynamical Forces/7(rho), Aerodynamical Torque/6(rho)

== system SixDOFSim/6 DOF Model Boeing 757 200/Forces and Moments Plane 1 ==
  Approach speed vA : Inport
  Angle of Attack Alpha : Inport  Port=2
  Slide Angle  beta : Inport  Port=3
  Throttel Position sigmaf : Inport  Port=4
  Lift Coeficcient CA : Inport  Port=5
  Drag Coefficient CW : Inport  Port=6
  Sideforce Coefficient CQ : Inport  Port=7
  CL : Inport  Port=8
  CM : Inport  Port=9
  CN : Inport  Port=10
  Air Density rho : Inport  Port=11
  Aerodynamical Forces : MATLAB Function  TreatAsAtomicUnit=on
  Aerodynamical Forces RA : Scope
      settings: ActiveDisplayYMinimum=-5.2551272052862361E+31  ActiveDisplayYMaximum=1.1237617783015539E+32
  Aerodynamical Torque : MATLAB Function  TreatAsAtomicUnit=on
  Sum : Sum  Inputs=++|
  Sum1 : Sum  Inputs=|++
  Thrust Force and Torque : MATLAB Function  TreatAsAtomicUnit=on
  Sum of external Forces : Outport
  Sum of external Torques : Outport  Port=2
  wires:
  Aerodynamical Forces/1(RA) -> Aerodynamical Forces RA/1, Sum1/1, Aerodynamical Torque/1(RA)
  Aerodynamical Torque/1(QA) -> Sum/2
  Sum1/1 -> Sum of external Forces/1
  Sum/1 -> Sum of external Torques/1
  Throttel Position sigmaf/1 -> Thrust Force and Torque/1(sigmaf)
  Thrust Force and Torque/1(Rf) -> Sum1/2
  Thrust Force and Torque/2(Qf) -> Sum/1
  Angle of Attack Alpha/1 -> Aerodynamical Forces/5(alpha)
  Slide Angle  beta/1 -> Aerodynamical Forces/6(beta)
  Approach speed vA/1 -> Aerodynamical Forces/4(vA), Aerodynamical Torque/5(vA)
  Lift Coeficcient CA/1 -> Aerodynamical Forces/1(CA)
  Drag Coefficient CW/1 -> Aerodynamical Forces/2(CW)
  Sideforce Coefficient CQ/1 -> Aerodynamical Forces/3(CQ)
  CL/1 -> Aerodynamical Torque/2(CL)
  CM/1 -> Aerodynamical Torque/3(CM)
  CN/1 -> Aerodynamical Torque/4(CN)
  Air Density rho/1 -> Aerodynamical Forces/7(rho), Aerodynamical Torque/6(rho)

== system SixDOFSim/6 DOF Model Boeing 757 200/Geometrical Coefficients Plain2 ==
  Approach Speed vA : Inport
  Angle of Attack alpha : Inport  Port=2
  Sideslip Angle beta : Inport  Port=3
  Rotation rates Omega : Inport  Port=4
  Elevator Angle eta : Inport  Port=5
  Rudder Angle zita : Inport  Port=6
  Airlon Angle xi : Inport  Port=7
  Geometrie Rotational Coefficients : MATLAB Function  TreatAsAtomicUnit=on
  Geometry Translational Coefficients : MATLAB Function  TreatAsAtomicUnit=on
  CA : Outport
  CW : Outport  Port=2
  CQ : Outport  Port=3
  CL : Outport  Port=4
  CM : Outport  Port=5
  CN : Outport  Port=6
  wires:
  Elevator Angle eta/1 -> Geometrie Rotational Coefficients/5(eta), Geometry Translational Coefficients/5(eta)
  Angle of Attack alpha/1 -> Geometrie Rotational Coefficients/2(alpha), Geometry Translational Coefficients/2(alpha)
  Geometrie Rotational Coefficients/1(CL) -> CL/1
  Geometry Translational Coefficients/3(CQ) -> CQ/1
  Geometrie Rotational Coefficients/3(CN) -> CN/1
  Approach Speed vA/1 -> Geometrie Rotational Coefficients/1(vA), Geometry Translational Coefficients/1(vA)
  Geometry Translational Coefficients/1(CA) -> CA/1
  Sideslip Angle beta/1 -> Geometrie Rotational Coefficients/3(beta), Geometry Translational Coefficients/3(beta)
  Rudder Angle zita/1 -> Geometrie Rotational Coefficients/6(zita), Geometry Translational Coefficients/6(zita)
  Geometry Translational Coefficients/2(CW) -> CW/1
  Rotation rates Omega/1 -> Geometrie Rotational Coefficients/4(Omega), Geometry Translational Coefficients/4(Omega)
  Geometrie Rotational Coefficients/2(CM) -> CM/1
  Airlon Angle xi/1 -> Geometrie Rotational Coefficients/7(xi)

== system SixDOFSim/6 DOF Model Boeing 757 200/Geometrical Coefficients Plane 1 ==
  Approach Speed vA : Inport
  Angle of Attack alpha : Inport  Port=2
  Sideslip Angle beta : Inport  Port=3
  Rotation rates Omega : Inport  Port=4
  Elevator Angle eta : Inport  Port=5
  Rudder Angle zita : Inport  Port=6
  Airlon Angle xi : Inport  Port=7
  Geometrie Rotational Coefficients : MATLAB Function  TreatAsAtomicUnit=on
  Geometry Translational Coefficients : MATLAB Function  TreatAsAtomicUnit=on
  CA : Outport
  CW : Outport  Port=2
  CQ : Outport  Port=3
  CL : Outport  Port=4
  CM : Outport  Port=5
  CN : Outport  Port=6
  wires:
  Elevator Angle eta/1 -> Geometrie Rotational Coefficients/5(eta), Geometry Translational Coefficients/5(eta)
  Angle of Attack alpha/1 -> Geometrie Rotational Coefficients/2(alpha), Geometry Translational Coefficients/2(alpha)
  Geometrie Rotational Coefficients/1(CL) -> CL/1
  Geometry Translational Coefficients/3(CQ) -> CQ/1
  Geometrie Rotational Coefficients/3(CN) -> CN/1
  Approach Speed vA/1 -> Geometrie Rotational Coefficients/1(vA), Geometry Translational Coefficients/1(vA)
  Geometry Translational Coefficients/1(CA) -> CA/1
  Sideslip Angle beta/1 -> Geometrie Rotational Coefficients/3(beta), Geometry Translational Coefficients/3(beta)
  Rudder Angle zita/1 -> Geometrie Rotational Coefficients/6(zita), Geometry Translational Coefficients/6(zita)
  Geometry Translational Coefficients/2(CW) -> CW/1
  Rotation rates Omega/1 -> Geometrie Rotational Coefficients/4(Omega), Geometry Translational Coefficients/4(Omega)
  Geometrie Rotational Coefficients/2(CM) -> CM/1
  Airlon Angle xi/1 -> Geometrie Rotational Coefficients/7(xi)

== system SixDOFSim/6 DOF Model Boeing 757 200/Motion model Plain1 ==
  Forces : Inport
  Torque : Inport  Port=2
  Wind Veloity : Inport  Port=3
  Dynamics : Subsystem
  ISA Atmosphere Model : aerolibatmos2/ISA Atmosphere Model  useExtended=off  action=None  custom=off  viscosityOut=off  g=9.80665  gamma=1.4  R=287.0531  L=0.0065  h_trop=11000  h_strat=20000  rho0=1.225  P0=101325  T0=288.15  h0=0  S=110.4  Tref=273.15  muref=1.716e-5
  Kinematics : Subsystem
  MATLAB Function : MATLAB Function  TreatAsAtomicUnit=on
  Mux : Mux  Inputs=2
  Terminator : Terminator
  Terminator1 : Terminator
  Terminator2 : Terminator
  Track and Aerodynamical Speed : MATLAB Function  TreatAsAtomicUnit=on
  Euler Angles (Phi) : Outport
  Position Down North East : Outport  Port=2
  Track Speed vk : Outport  Port=3
  Approach Speed (vA) : Outport  Port=4
  Angle of Attack (alpha) : Outport  Port=5
  Slidiing Angle (beta) : Outport  Port=6
  Rotation Rate Omega : Outport  Port=7
  Air Density rho : Outport  Port=8
  "Course Angles (gamma;chsi) " : Outport  Port=9
  Translational Speed V : Outport  Port=10
  wires:
  Torque/1 -> Dynamics/2(Torque)
  Kinematics/1(Euler Angle (Phi)) -> Track and Aerodynamical Speed/1(Phi), Dynamics/3(Euler Angles( Phi)), Euler Angles (Phi)/1  "Euler Angles (Phi)"
  Kinematics/2(P_erdfest) -> Position Down North East/1, MATLAB Function/1(P_e)  "(P_erdfest)"
  Dynamics/2(Translational Speed V) -> Kinematics/2(V), Translational Speed V/1, Track and Aerodynamical Speed/2(V)  "V"
  Forces/1 -> Dynamics/1(Forces)
  Dynamics/1(Rotation Rate Omega) -> Rotation Rate Omega/1, Kinematics/1(Omega)
  Wind Veloity/1 -> Track and Aerodynamical Speed/3(Vw_geod)
  MATLAB Function/1(h) -> ISA Atmosphere Model/1
  ISA Atmosphere Model/4 -> Air Density rho/1
  Track and Aerodynamical Speed/1(vk) -> Track Speed vk/1
  ISA Atmosphere Model/1 -> Terminator/1
  ISA Atmosphere Model/2 -> Terminator1/1
  ISA Atmosphere Model/3 -> Terminator2/1
  Track and Aerodynamical Speed/2(vA) -> Approach Speed (vA)/1
  Track and Aerodynamical Speed/3(alpha) -> Angle of Attack (alpha)/1
  Track and Aerodynamical Speed/4(beta) -> Slidiing Angle (beta)/1
  Mux/1 -> "Course Angles (gamma;chsi) "/1
  Track and Aerodynamical Speed/5(gamma) -> Mux/1
  Track and Aerodynamical Speed/6(chsi) -> Mux/2

== system SixDOFSim/6 DOF Model Boeing 757 200/Motion model Plain2  ==
  Forces : Inport
  Torque : Inport  Port=2
  Wind Veloity : Inport  Port=3
  Dynamics : Subsystem
  ISA Atmosphere Model : aerolibatmos2/ISA Atmosphere Model  useExtended=off  action=None  custom=off  viscosityOut=off  g=9.80665  gamma=1.4  R=287.0531  L=0.0065  h_trop=11000  h_strat=20000  rho0=1.225  P0=101325  T0=288.15  h0=0  S=110.4  Tref=273.15  muref=1.716e-5
  Kinematics : Subsystem
  MATLAB Function : MATLAB Function  TreatAsAtomicUnit=on
  Mux : Mux  Inputs=2
  Terminator : Terminator
  Terminator1 : Terminator
  Terminator2 : Terminator
  Track and Aerodynamical Speed : MATLAB Function  TreatAsAtomicUnit=on
  Euler Angles (Phi) : Outport
  Position Down North East : Outport  Port=2
  Track Speed vk : Outport  Port=3
  Approach Speed (vA) : Outport  Port=4
  Angle of Attack (alpha) : Outport  Port=5
  Slidiing Angle (beta) : Outport  Port=6
  Rotation Rate Omega : Outport  Port=7
  Air Density rho : Outport  Port=8
  "Course Angles (gamma;chsi) " : Outport  Port=9
  Translational Speed V : Outport  Port=10
  wires:
  Torque/1 -> Dynamics/1(Torque)
  Kinematics/1(Euler Angle (Phi)) -> Track and Aerodynamical Speed/1(Phi), Dynamics/3(Euler Angles( Phi)), Euler Angles (Phi)/1  "Euler Angles (Phi)"
  Kinematics/2(P_erdfest) -> Position Down North East/1, MATLAB Function/1(P_e)  "(P_erdfest)"
  Dynamics/2(Translational Speed V) -> Kinematics/2(V), Translational Speed V/1, Track and Aerodynamical Speed/2(V)  "V"
  Dynamics/1(Rotation Rate Omega) -> Rotation Rate Omega/1, Kinematics/1(Omega)
  Wind Veloity/1 -> Track and Aerodynamical Speed/3(Vw_geod)
  MATLAB Function/1(h) -> ISA Atmosphere Model/1
  ISA Atmosphere Model/4 -> Air Density rho/1
  Track and Aerodynamical Speed/1(vk) -> Track Speed vk/1
  ISA Atmosphere Model/1 -> Terminator/1
  ISA Atmosphere Model/2 -> Terminator1/1
  ISA Atmosphere Model/3 -> Terminator2/1
  Track and Aerodynamical Speed/2(vA) -> Approach Speed (vA)/1
  Track and Aerodynamical Speed/3(alpha) -> Angle of Attack (alpha)/1
  Track and Aerodynamical Speed/4(beta) -> Slidiing Angle (beta)/1
  Mux/1 -> "Course Angles (gamma;chsi) "/1
  Track and Aerodynamical Speed/5(gamma) -> Mux/1
  Track and Aerodynamical Speed/6(chsi) -> Mux/2
  Forces/1 -> Dynamics/2(Forces)
